simulink model "SITRA_Traffic_Hardware"  (R2026a)
settings: Solver=FixedStepDiscrete  StartTime=0  StopTime=600  FixedStep=1
model workspace (MAT data in the model file):
  T = 600
  cycleLength = 63
  dt = 1
  maxGreen = 30
  minGreen = 12
  normalDemand = [0.1 0.07 0.05]
  surgeDemand = [0.3 0.07 0.05]
  surgeEnd = 400
  surgeStart = 200
  yellowTime = 3
Description:
  | S1 architecture for the SITRA traffic-management and power-electronics implementation roadmap.
  | 
  | Reference traffic network: HopeCollege, Kalapatti, Airport -> SITRA -> Goldwins.
  | Frozen Part 8 MPC is the supervisory reference controller.
  | S1 contains architecture only; detailed dynamics are implemented later.
  | 
  | Simulation parameters:
  | dt = 1.0 s
  | T = 600.0 s
  | Cycle = 63.0 s
  | Yellow/Clearance = 3.0 s
  | Minimum green = 12.0 s
  | Maximum green = 30.0 s
  | Normal demand = [0.10 0.07 0.05] veh/s
  | Surge demand = [0.30 0.07 0.05] veh/s
  | Surge interval = 200.0 to 400.0 s
settings Model: Creator=Sreedev  LastModifiedBy=saisi

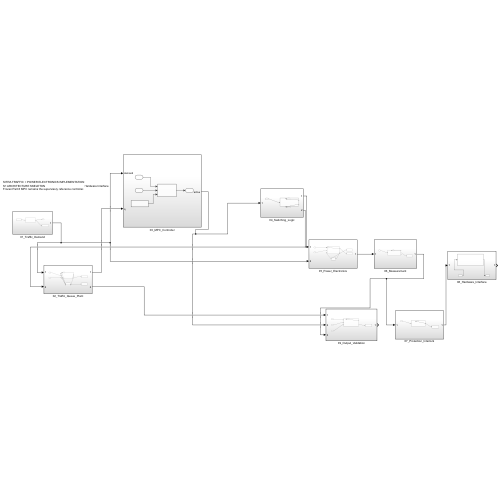
[thumbnail: Simulink's stored preview of the top-level diagram]
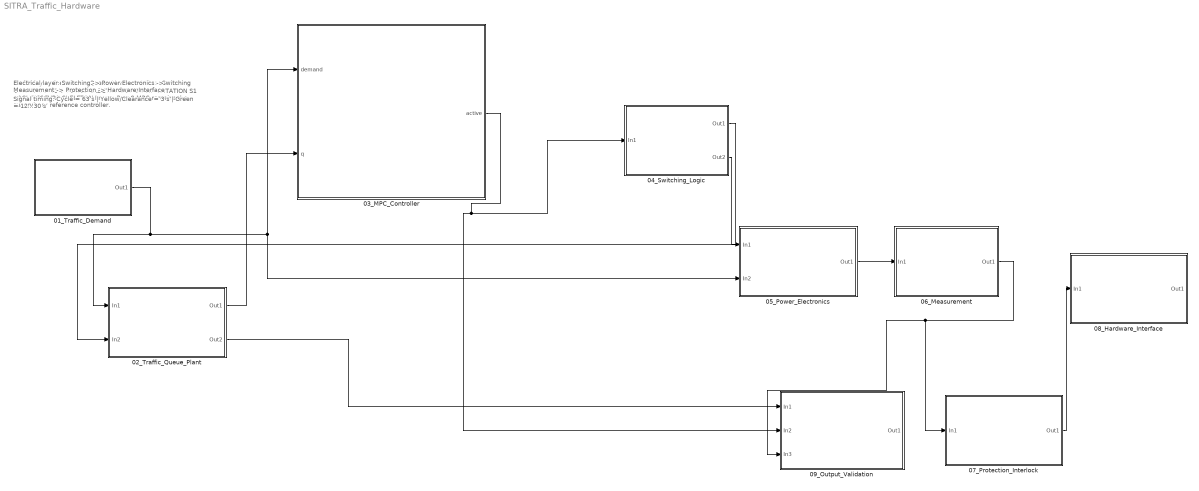
== system SITRA_Traffic_Hardware ==
  note: SITRA TRAFFIC + POWER ELECTRONICS IMPLEMENTATION
      | S1 ARCHITECTURE SKELETON
      | Frozen Part 8 MPC remains the supervisory reference controller.
  note: Traffic layer:
      | Demand -> Queue Plant -> MPC -> Switching
  note: Electrical layer:
      | Switching -> Power Electronics -> Measurement -> Protection -> Hardware Interface
  note: Signal timing:
      | Cycle = 63 s | Yellow/Clearance = 3 s | Green = 12...30 s
  01_Traffic_Demand : Subsystem
  02_Traffic_Queue_Plant : Subsystem
  03_MPC_Controller : Subsystem
  04_Switching_Logic : Subsystem
  05_Power_Electronics : Subsystem
  06_Measurement : Subsystem
  07_Protection_Interlock : Subsystem
  08_Hardware_Interface : Subsystem
  09_Output_Validation : Subsystem
  wires:
  01_Traffic_Demand/1(Out1) -> 05_Power_Electronics/2(In2), 03_MPC_Controller/1(demand), 02_Traffic_Queue_Plant/1(In1)
  02_Traffic_Queue_Plant/1(Out1) -> 03_MPC_Controller/2(q)
  03_MPC_Controller/1(active) -> 09_Output_Validation/2(In2), 04_Switching_Logic/1(In1)
  04_Switching_Logic/1(Out1) -> 02_Traffic_Queue_Plant/2(In2)
  04_Switching_Logic/2(Out2) -> 05_Power_Electronics/1(In1)
  05_Power_Electronics/1(Out1) -> 06_Measurement/1(In1)
  06_Measurement/1(Out1) -> 09_Output_Validation/3(In3), 07_Protection_Interlock/1(In1)
  07_Protection_Interlock/1(Out1) -> 08_Hardware_Interface/1(In1)
  02_Traffic_Queue_Plant/2(Out2) -> 09_Output_Validation/1(In1)

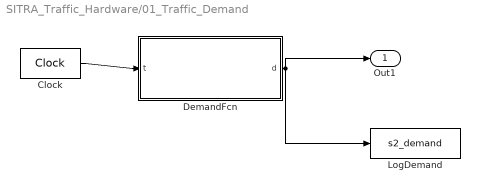
== system SITRA_Traffic_Hardware/01_Traffic_Demand ==
  Clock : DigitalClock
  DemandFcn : MATLAB Function  TreatAsAtomicUnit=on
  LogDemand : ToWorkspace  VariableName=s2_demand  SampleTime=1
  Out1 : Outport
  wires:
  Clock/1 -> DemandFcn/1(t)
  DemandFcn/1(d) -> Out1/1, LogDemand/1

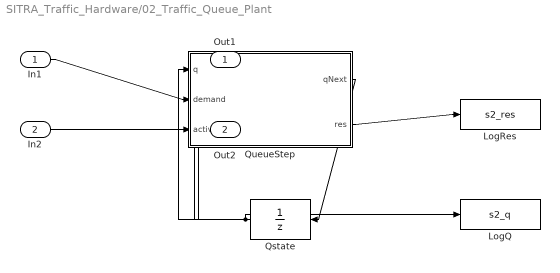
== system SITRA_Traffic_Hardware/02_Traffic_Queue_Plant ==
  In1 : Inport
  In2 : Inport  Port=2
  LogQ : ToWorkspace  VariableName=s2_q  SampleTime=1
  LogRes : ToWorkspace  VariableName=s2_res  SampleTime=1
  Qstate : UnitDelay  InitialCondition=zeros(4,1)
  QueueStep : MATLAB Function  TreatAsAtomicUnit=on
  Out1 : Outport
  Out2 : Outport  Port=2
  wires:
  Qstate/1 -> QueueStep/1(q), Out1/1, Out2/1, LogQ/1
  In1/1 -> QueueStep/2(demand)
  In2/1 -> QueueStep/3(active)
  QueueStep/1(qNext) -> Qstate/1
  QueueStep/2(res) -> LogRes/1

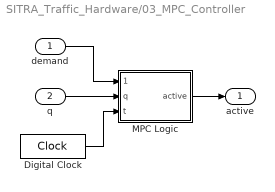
== system SITRA_Traffic_Hardware/03_MPC_Controller ==
  demand : Inport
  q : Inport  Port=2
  Digital Clock : DigitalClock
  MPC Logic : MATLAB Function  TreatAsAtomicUnit=on
  active : Outport
  wires:
  demand/1 -> MPC Logic/1(demand)
  q/1 -> MPC Logic/2(q)
  Digital Clock/1 -> MPC Logic/3(t)
  MPC Logic/1(active) -> active/1

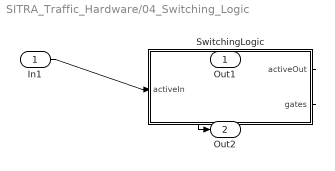
== system SITRA_Traffic_Hardware/04_Switching_Logic ==
  In1 : Inport
  SwitchingLogic : MATLAB Function  TreatAsAtomicUnit=on
  Out1 : Outport
  Out2 : Outport  Port=2
  wires:
  In1/1 -> SwitchingLogic/1(activeIn)
  SwitchingLogic/1(activeOut) -> Out1/1
  SwitchingLogic/2(gates) -> Out2/1

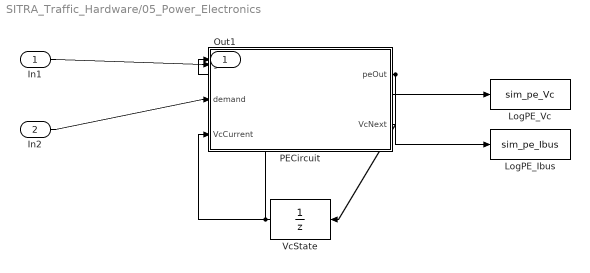
== system SITRA_Traffic_Hardware/05_Power_Electronics ==
  In1 : Inport
  In2 : Inport  Port=2
  LogPE_Ibus : ToWorkspace  VariableName=sim_pe_Ibus  SampleTime=1
  LogPE_Vc : ToWorkspace  VariableName=sim_pe_Vc  SampleTime=1
  PECircuit : MATLAB Function  TreatAsAtomicUnit=on
  VcState : UnitDelay  InitialCondition=zeros(1,4)
  Out1 : Outport
  wires:
  In1/1 -> PECircuit/1(gates)
  In2/1 -> PECircuit/2(demand)
  VcState/1 -> PECircuit/3(VcCurrent), LogPE_Vc/1
  PECircuit/2(VcNext) -> VcState/1
  PECircuit/1(peOut) -> Out1/1, LogPE_Ibus/1

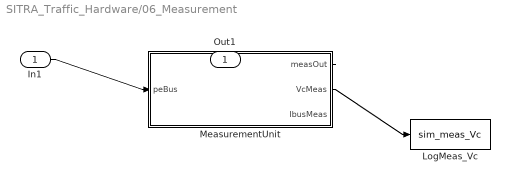
== system SITRA_Traffic_Hardware/06_Measurement ==
  In1 : Inport
  LogMeas_Vc : ToWorkspace  VariableName=sim_meas_Vc  SampleTime=1
  MeasurementUnit : MATLAB Function  TreatAsAtomicUnit=on
  Out1 : Outport
  wires:
  In1/1 -> MeasurementUnit/1(peBus)
  MeasurementUnit/1(measOut) -> Out1/1
  MeasurementUnit/2(VcMeas) -> LogMeas_Vc/1

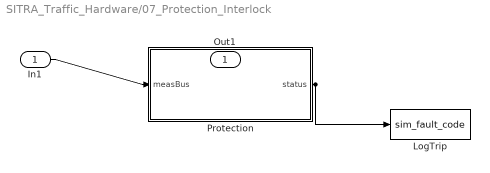
== system SITRA_Traffic_Hardware/07_Protection_Interlock ==
  In1 : Inport
  LogTrip : ToWorkspace  VariableName=sim_fault_code  SampleTime=1
  Protection : MATLAB Function  TreatAsAtomicUnit=on
  Out1 : Outport
  wires:
  In1/1 -> Protection/1(measBus)
  Protection/1(status) -> Out1/1, LogTrip/1

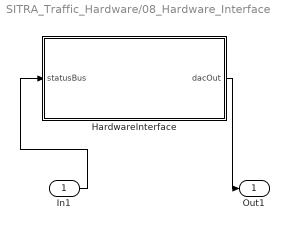
== system SITRA_Traffic_Hardware/08_Hardware_Interface ==
  In1 : Inport
  HardwareInterface : MATLAB Function  TreatAsAtomicUnit=on
  Out1 : Outport
  wires:
  In1/1 -> HardwareInterface/1(statusBus)
  HardwareInterface/1(dacOut) -> Out1/1

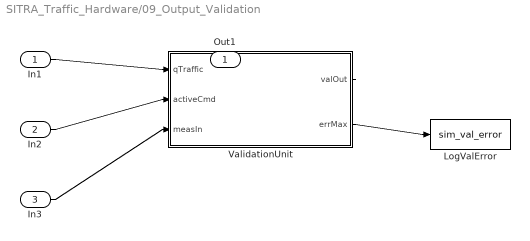
== system SITRA_Traffic_Hardware/09_Output_Validation ==
  In1 : Inport
  In2 : Inport  Port=2
  In3 : Inport  Port=3
  LogValError : ToWorkspace  VariableName=sim_val_error  SampleTime=1
  ValidationUnit : MATLAB Function  TreatAsAtomicUnit=on
  Out1 : Outport
  wires:
  In1/1 -> ValidationUnit/1(qTraffic)
  In2/1 -> ValidationUnit/2(activeCmd)
  In3/1 -> ValidationUnit/3(measIn)
  ValidationUnit/1(valOut) -> Out1/1
  ValidationUnit/2(errMax) -> LogValError/1

== matlab function SITRA_Traffic_Hardware/01_Traffic_Demand/DemandFcn ==
  data: t input; d output
function d = demandProfile(t)
% Normal / surge demand [B1 B2 B3] veh/s (matches Part 8)
normalD = [0.10 0.07 0.05];
surgeD  = [0.30 0.07 0.05];
if t >= 200 && t < 400
    d = surgeD;
else
    d = normalD;
end
end

== matlab function SITRA_Traffic_Hardware/02_Traffic_Queue_Plant/QueueStep ==
  data: q input; qNext output; demand input; active input; res output
function [qNext, res] = queueStep(q, demand, active)
% Four-branch traffic queue plant

% Ensure column vectors
q = q(:);
demand = demand(:);

% Branch capacities
cap = [0.65; 0.35; 0.25; 0.45];

dt = 1;

% Arrivals and departures
arr = [demand; 0];
dep = zeros(4,1);

a = round(active);

if a >= 1 && a <= 3
    dep(a) = min(cap(a), q(a)/dt);
    arr(4) = dep(a);
end

dep(4) = min(cap(4), q(4)/dt);

% Queue update
qNext = max(zeros(4,1), q + dt*(arr-dep));

% Conservation residual
res = arr-dep-(qNext-q)/dt;

end

== matlab function SITRA_Traffic_Hardware/03_MPC_Controller/MPC Logic ==
  data: demand input; active output; q input; t input
function active = fcn(demand, q, t)
% SITRA MPC Traffic Signal Controller
% Inputs:
% demand = traffic demand [B1 B2 B3]
% q      = queue lengths [B1 B2 B3 B4]
% t      = simulation time

% Ensure row vectors
demand = reshape(demand,1,3);
q = reshape(q,1,4);

% Controller parameters
n = 3;
yellow = 3;
cycleLength = 63;
minGreen = 12;
maxGreen = 30;

totalGreen = cycleLength - n*yellow;

% Initial green allocation
base = minGreen*ones(1,n);
remaining = totalGreen - sum(base);

% Predictive priority score
score = max(q(1:n),0) + 10*max(demand,0);
score(2:3) = score(2:3) + 0.25;

% Allocate remaining green time
greenTimes = base;

for s = 1:round(remaining)

    room = maxGreen - greenTimes;
    [m,idx] = max(score .* (room > 1e-12));

    if m <= 0
        break;
    end

    greenTimes(idx) = greenTimes(idx) + 1;
    score(idx) = score(idx)*0.985 + 1e-12;

end

% Correct rounding mismatch
diffGreen = totalGreen - sum(greenTimes);

while abs(diffGreen) > 1e-12

    if diffGreen > 0
        room = maxGreen-greenTimes;
        [mx,idx] = max(room);

        if mx <= 0
            break;
        end

        add = min(diffGreen,mx);
        greenTimes(idx) = greenTimes(idx)+add;

    else
        room = greenTimes-minGreen;
        [mx,idx] = max(room);

        if mx <= 0
            break;
        end

        sub = min(-diffGreen,mx);
        greenTimes(idx) = greenTimes(idx)-sub;
    end

    diffGreen = totalGreen-sum(greenTimes);

end

% Determine active traffic branch
tau = mod(t,cycleLength);
current = 0;
active = 0;

for p = 1:n

    gEnd = current + greenTimes(p);
    yEnd = gEnd + yellow;

    if tau >= current && tau < gEnd
        active = p;
        return;

    elseif tau >= gEnd && tau < yEnd
        active = 0;
        return;
    end

    current = yEnd;

end

end

== matlab function SITRA_Traffic_Hardware/04_Switching_Logic/SwitchingLogic ==
  data: activeIn input; activeOut output; gates output
function [activeOut, gates] = switchingLogic(activeIn)
% Generates isolated gate drive pulses [g1 g2 g3] with clearance dead-time
a = round(activeIn);
activeOut = double(a);
gates = zeros(1,3);
if a >= 1 && a <= 3
    gates(a) = 1.0;
end
% Interlock assert: at most one gate high
assert(sum(gates) <= 1, 'Shoot-through fault: Multiple gates active!');
end

== matlab function SITRA_Traffic_Hardware/05_Power_Electronics/PECircuit ==
  data: gates input; peOut output; demand input; VcCurrent input; VcNext output
function [peOut, VcNext] = peCircuitStep(gates, demand, VcCurrent)
% Complete Equivalent Power Electronic Circuit Update (1 s step)
% Parameters:
C = [1.0 1.0 1.0 1.0];             % Capacitances [F]
I_sat = [0.65 0.35 0.25 0.45];     % Road saturation current limits [A]
R_on = 0.01;                       % MOSFET on-resistance [Ohm]
dt = 1.0;
g = reshape(gates, 1, 3);
d = reshape(demand, 1, 3);
vc = reshape(VcCurrent, 1, 4);

% Input currents from demand converters
i_arr = zeros(1,4);
i_arr(1:3) = d;

% Semiconductor switch conduction
i_dep = zeros(1,4);
for b = 1:3
    if g(b) > 0.5
        i_dep(b) = min(I_sat(b), vc(b)/dt);
    end
end

% SITRA Junction Common DC Bus (Summing node)
i_bus = sum(i_dep(1:3));
i_arr(4) = i_bus;

% Downstream bottleneck current sink (Goldwins exit)
i_dep(4) = min(I_sat(4), vc(4)/dt);

% KCL integration with clamping diodes (Vc >= 0)
VcNext = max(zeros(1,4), vc + (dt ./ C) .* (i_arr - i_dep));

% Conduction power loss and stored energy
p_loss = sum(i_dep(1:3).^2) * R_on;
e_tot = 0.5 * sum(C .* (vc.^2));

% Pack electrical output vector: [Vc(1..4), I_in(1..4), I_dep(1..4), I_bus, p_loss, e_tot]
peOut = [vc, i_arr, i_dep, i_bus, p_loss, e_tot];
end

== matlab function SITRA_Traffic_Hardware/06_Measurement/MeasurementUnit ==
  data: peBus input; measOut output; VcMeas output; IbusMeas output
function [measOut, VcMeas, IbusMeas] = measurementUnit(peBus)
% High-precision voltage & current instrumentation
vc = peBus(1:4);
i_bus = peBus(9);
p_loss = peBus(10);
e_tot = peBus(11);

VcMeas = vc;
IbusMeas = i_bus;
measOut = [vc, i_bus, e_tot, p_loss];
end

== matlab function SITRA_Traffic_Hardware/07_Protection_Interlock/Protection ==
  data: measBus input; status output
function status = protectionInterlock(measBus)
% Fault and protection monitor
vc = measBus(1:4);
i_bus = measBus(5);

% Over-voltage / severe congestion threshold (e.g., 20 V / 20 vehicles)
overVoltageTrip = any(vc > 20.0);
bottleneckWarn = (i_bus >= 0.449);

% 0 = Normal, 1 = Warning, 2 = Trip
faultCode = 0.0;
if overVoltageTrip
    faultCode = 2.0;
elseif bottleneckWarn
    faultCode = 1.0;
end
status = [faultCode, double(overVoltageTrip), double(bottleneckWarn)];
end

== matlab function SITRA_Traffic_Hardware/08_Hardware_Interface/HardwareInterface ==
  data: statusBus input; dacOut output
function dacOut = hardwareInterface(statusBus)
% Scales physical circuit protection and status for 0-3.3V DSP / GPIO Channels
faultCode = statusBus(1);
% Opto-isolated GPIO signals (3.3 V active high)
tripGpio = double(faultCode >= 2.0) * 3.3;
warnGpio = double(faultCode == 1.0) * 3.3;
dacOut = [statusBus, tripGpio, warnGpio];
end

== matlab function SITRA_Traffic_Hardware/09_Output_Validation/ValidationUnit ==
  data: qTraffic input; valOut output; activeCmd input; measIn input; errMax output
function [valOut, errMax] = validationUnit(qTraffic, activeCmd, measIn)
% Real-time verification of traffic-circuit mathematical equivalence
q = reshape(qTraffic, 1, 4);
vc = reshape(measIn(1:4), 1, 4);
err = abs(vc - q);
errMax = max(err);
valOut = [err, double(errMax < 1e-9), double(activeCmd)];
end
